simulink model "ex10_I2C"  (Simulink 7.6)
settings: Solver=FixedStepDiscrete  SolverMode=SingleTasking  StartTime=0.0  StopTime=inf  FixedStep=0.001  RelTol=1e-3
libraries: dsPICdrivers x8, simulink x2, commutil2 x1
settings Model: Creator=Lior  LastModifiedBy=Lior  BufferReuse=off
settings OptimizationCC: BlockReduction=off  InlineParams=on  BufferReuse=off  OptimizeModelRefInitCode=on  LifeSpan=1
settings HardwareCC: ProdBitPerInt=16  ProdBitPerPointer=16  ProdEndianess=LittleEndian  ProdWordSize=16  ProdHWDeviceType=16-bit Generic
settings RTWCC: SystemTargetFile=dspic.tlc  MakeCommand=make_CreateMPLAB  TemplateMakefile=dspic_pic30_gcc.tmf  PostCodeGenCommand=dsPIC_Compile()  Description=Embedded Target for Microchip dsPIC (real-time)  ProcessScript=dspic_make_rtw_hook
settings CodeAppCC: IgnoreCustomStorageClasses=off
settings STFCustomTargetCC: IncludeMdlTerminateFcn=off  CombineOutputUpdateFcns=on  SuppressErrorStatus=on  ERTCustomFileBanners=on  SupportContinuousTime=off  SupportNonInlinedSFcns=off  SystemTargetFile=dspic.tlc
settings ERTTargetCC: MultiwordLength=2048  ParMdlRefBuildCompliant=off  CompOptLevelCompliant=off  IncludeMdlTerminateFcn=off  SuppressErrorStatus=on  ERTFirstTimeCompliant=off  ModelStepFunctionPrototypeControlCompliant=off  CPPClassGenCompliant=off  ExtModeMexFile=ext_serial_win32_comm  InlinedParameterPlacement=NonHierarchical  ERTSrcFileBannerTemplate=dsPIC_code_template.cgt  ERTHdrFileBannerTemplate=dsPIC_code_template.cgt  ERTDataSrcFileTemplate=dsPIC_code_template.cgt  ERTDataHdrFileTemplate=dsPIC_code_template.cgt  ERTCustomFileTemplate=dsPIC_main.tlc  ConvertIfToSwitch=off
settings CustomProperty: DataType=string  Value=C:\PROGRA~1\MATLAB\R2010b\bin\win64\gmake
settings SimEventsCC: propDiagAttribOutput=1  propDiagFcnCallOutput=1  propDiagStatOutput=0

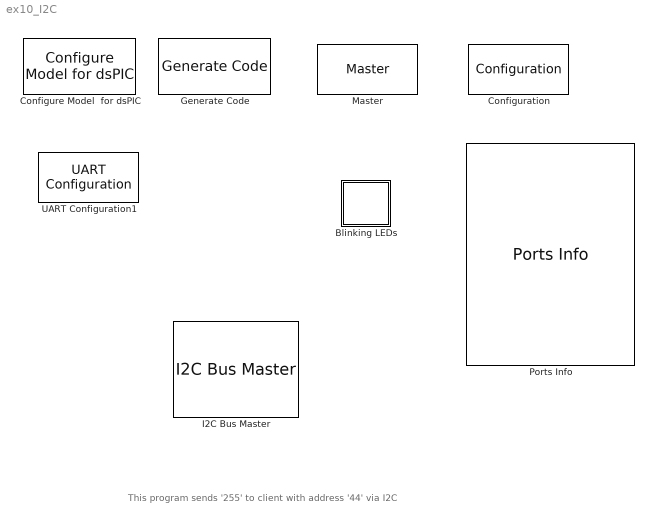
== system ex10_I2C ==
  note: This program sends '255' to client with address '44' via I2C
  Blinking LEDs : Subsystem
  Configuration : dsPICdrivers/Configuration  SystemSampleTime=-1  double64=off
  Configure Model  for dsPIC : dsPICdrivers/Simulink Configuration/Configure Model  for dsPIC
  Generate Code : dsPICdrivers/Simulink Configuration/Generate Code
  I2C Bus Master : dsPICdrivers/BUS I2C/I2C Bus Master  Tag=dsPIC_I2C_Master  NumI2C=2  AltI2C=off  Sequence='S A88 W255 P'  InitializeOnceOnly=When PIC is initialized (only once)  Enable=on  WaitAfterEnable=1  Disable=on  AdressNbrBits=7 bits  I2CBusFreq=360  SlewRate=off  SMBUSThreshold=off  OutputErrorFlag=off  SampleTime=0.1  OrderingInOutPopup=None  Info=Fscl = 20.0605 KHz
  Master : dsPICdrivers/Master  Tag=dsPIC_MASTER  Priority=1  TimeStepType=Timer1  picType=33fJ256GP710A  fcy=7375000  Quartz_33f=8e6  PLLActive_33f=on  fcyDesired_33f=7.37e6  tmr1="[1  7374  0]"  tmr1Info="Time Step : 0.001  ;   Error : 0%  PR1=7374"  tmr2345="[0  0  0  0  0  0  0  0]"  tmr2345cfg=[-1 -1 -1 -1 -1 -1 -1 -1]  IOautoConf=on  typePort="[ 0   0  20  20   0   0   0   0   0   0   0   0   0   0   0   0   0   0   0   0   0   0   0   0   0   0   0   0   0   0   0   0   0   0   0   0   0   0   0   0   0   0   0   0   0   0   0   0   0   0   0   0   0   0   0   0   0   0   0   0   0   0   0   0   0  10  10  10  10   0   0   0   0   0   0   0   0   0   0   0   0   0   0   0   4   0   0   0   0   0   0   0   0   0   0   0   0   0   0   0   0   0   0   0   0   0   0   0   0   0   0   0 ]"  TRIS="[ 65535  65535  65535  65535  65505  65535  65535 ]"  ADPCFG=503316480  MasterBusyPort=None  MasterOverloadPort=None  FOSC=Quartz (XT - HS)  ClockSwitchMonitor=Clock switching enabled only  TempProtection_33f=TEMP_ON  FPBOR=<empty>  PWRT=disable  MCLR=<empty>  ICD=ICS_PGD1  JTAGEN=JTAGEN_OFF  PowerSave=off  OverrideFcy=off  NewFcy=1e6  PR2345="[65535  65535  65535  65535  65535  65535  65535  65535]"
  Ports Info : dsPICdrivers/Ports Info  Tag=dsPIC_PortInfo
  UART Configuration1 : dsPICdrivers/Serial PORT/UART Configuration  Tag=dsPIC_config_UART  Priority=2  UART=2  proposed_BAUD=115200  BAUD=115200  ALT_TX_RX=on  InterruptTxWhen=When Transmit Buffer is empty  TXInterruptPri=1  TxBufferSize=32  TXEN=off  InterruptRxWhen=When Receive Buffer is full (contain 4 characters)  RXInterruptPri=2  RxBufferSize=32  DoNotImplementRxInterrupt=off  DoNotImplementTxInterrupt=off  UxBRG=3  Info="UxBRG = 3   ||  Real Baud : 115234   ||  % error : 0.029839  ||  max 11.5234 Bytes / Step"  RealBaud=0  ERROR=0.029839  BYTES_STEP=11.5234

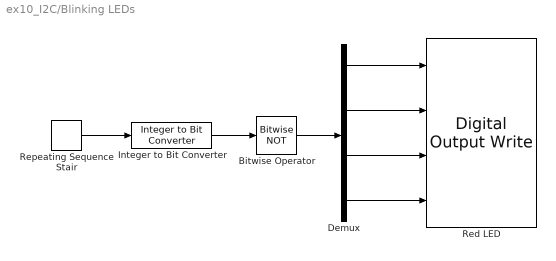
== system ex10_I2C/Blinking LEDs ==
  Bitwise Operator : simulink/Logic and Bit Operations/Bitwise Operator  logicop=NOT  UseBitMask=off  BitMask=bin2dec('11011001')  BitMaskRealWorld=Stored Integer
  Demux : Demux
  Integer to Bit Converter : commutil2/Integer to Bit Converter  nbits=4  signedInputValues=Unsigned  bitOrder=MSB first  outDtype=boolean
  Red LED : dsPICdrivers/Digital I//O/Digital Output Write  Tag=dsPIC_Digital_Output  Priority=5  PORT=E  Pin=[1 2 3 4]  Simultaneous=on  OrderingInOutPopup=None
  Repeating Sequence Stair : simulink/Sources/Repeating Sequence Stair  SystemSampleTime=-1  OutValues=[0 1 3 7 14 12 8 ].'  tsamp=0.1  OutMin=[]  OutMax=[]  OutDataTypeStr=uint8  OutputDataTypeScalingMode=uint8  OutDataType=fixdt(0,8)  ConRadixGroup=Best Precision: Vector-wise  OutScaling=2^-12
  wires:
  Repeating Sequence Stair/1 -> Integer to Bit Converter/1
  Integer to Bit Converter/1 -> Bitwise Operator/1
  Demux/1 -> Red LED/1
  Demux/2 -> Red LED/2
  Demux/3 -> Red LED/3
  Demux/4 -> Red LED/4
  Bitwise Operator/1 -> Demux/1
